simulink model "NBMS_CCCV"  (R2026b)
settings: Solver=FixedStepDiscrete  StopTime=25  FixedStep=0.1
undefined symbols (not defined in the file): CAL_CC_END_DEBOUNCE_TIMER, CAL_CC_END_THRSH, CAL_CHRG_CC_CURRENT_LIMIT, CAL_CHRG_CV_CURRENT_LIMIT, CAL_CHRG_VOLT_LIMIT, CAL_CV_COMPLETE_TIMER, CAL_CV_END_DEBOUNCE_TIMER, CAL_CV_END_THRSH, CAL_CV_WAIT_TIMER, CAL_DD_REVIVAL_CCL, X_CCL_CONT_SAFETY_PACK, Y_CCL_CONT_SAFETY_PACK
settings Model: Creator=hp  LastModifiedBy=rathi
settings OptimizationCC: DefaultParameterBehavior=Inlined  DifferentSizesBufferReuse=on  EfficientTunableParamExpr=on  EnhancedBackFolding=on  OptimizationCustomize=off  OptimizeBlockOrder=speed  PassReuseOutputArgsAs=Individual arguments  RemoveInternalMemoryZeroInit=on  RemoveRootLevelIOMemoryZeroInit=on
settings DebuggingCC: ParameterTunabilityLossMsg=error
settings SFSimCC: MATLABDynamicMemAlloc=off
settings RTWCC: Description=Embedded Coder  GenCodeOnly=on  PackageGeneratedCodeAndArtifacts=on  SystemTargetFile=ert.tlc  TemplateMakefile=ert_default_tmf
settings CodeAppCC: ForceParamTrailComments=on  IgnoreCustomStorageClasses=off  InsertBlockDesc=on  OperatorAnnotations=on  SFDataObjDesc=on  SimulinkDataObjDesc=on
settings ERTTargetCC: DynamicArrayContainerType=coder::array  GenerateSampleERTMain=on
settings ConfigComp: DVDefectChecker=on  DVDetectOutOfBounds=on  DVHarnessSource=Signal Editor  DVModelReferenceHarness=on  DVTestSuiteOptimization=Auto

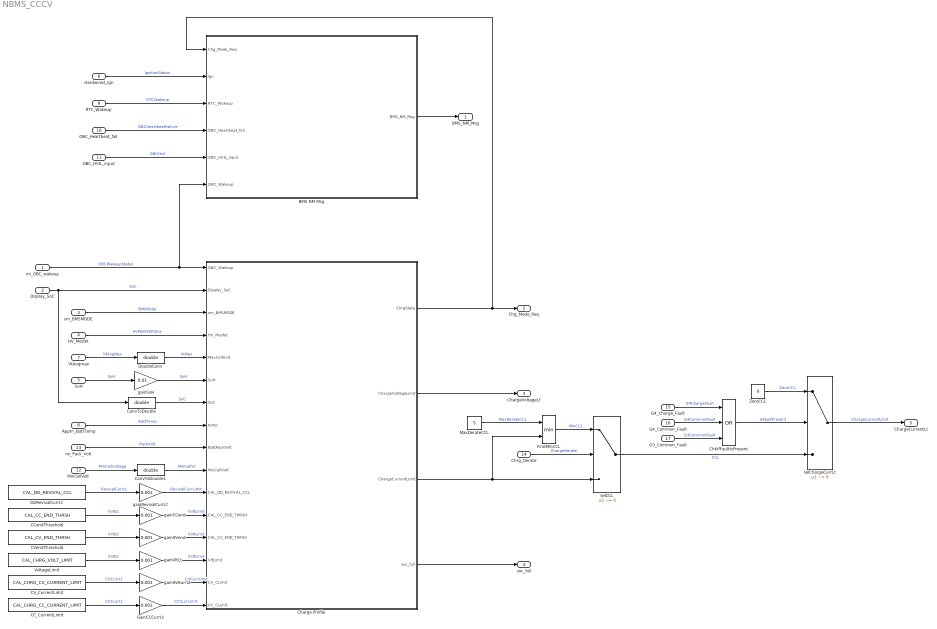
== system NBMS_CCCV ==
  mi_OBC_wakeup : Inport  OutDataTypeStr=Enum: OBC_E
  Display_SoC : Inport  Port=2  OutDataTypeStr=uint8
  sm_BMSMODE : Inport  Port=3  OutDataTypeStr=Enum: BMS_MODE_E
  HV_Mosfet : Inport  Port=4  OutDataTypeStr=Enum: BMS_HVMosfet_STS_E
  SoH : Inport  Port=5  OutDataTypeStr=double
  AppIn_BattTemp : Inport  Port=6  OutDataTypeStr=double
  VtAvgmax : Inport  Port=7  OutDataTypeStr=fixdt(1,16,0.001,0)
  Hardwired_Ign : Inport  Port=8  OutDataTypeStr=boolean
  RTC_Wakeup : Inport  Port=9  OutDataTypeStr=boolean
  OBC_Heartbeat_fail : Inport  Port=10  OutDataTypeStr=boolean
  OBC_HVIL_input : Inport  Port=11  OutDataTypeStr=boolean
  MinCellVolt : Inport  Port=12  OutDataTypeStr=fixdt(1,16,0.001,0)
  mi_Pack_Volt : Inport  Port=13  OutDataTypeStr=double
  Chrg_Derate : Inport  Port=14  OutDataTypeStr=boolean
  G4_Charge_Fault : Inport  Port=15  OutDataTypeStr=boolean
  G4_Common_Fault : Inport  Port=16  OutDataTypeStr=boolean
  G3_Common_Fault : Inport  Port=17  OutDataTypeStr=boolean
  BMS NM Msg : Stateflow chart  TreatAsAtomicUnit=on
      settings: PortSchema="{\"entries\":[{\"content\":{\"sides\":[{\"content\":{\"connectorIds\":[\"In1\",\"In2\",\"In3\",\"In5\",\"In6\",\"In4\"]},\"type\":\"ConnectorPlacement.EquallySpacedRectSide\",\"uuid\":\"e6ae22f8-5427-4fcf-97e7-049847468580\"},{\"content\":{\"connectorIds\":[\"Out1\"],\"side\":\"RIGHT\"},\"type\":\"ConnectorPlacement.EquallySpacedRectSide\",\"uuid\":\"de67337b-b27c-48bc-b99a-9da25b5b262a\"},{\"content\":{\"side\":\"TOP\"},\"type\":\"ConnectorPlacement.EquallySpacedRectSide\",\"uuid\":\"908dc17d-6a46-4063-b5b5-053b8a862aa1\"}]},\"type\":\"ConnectorPlacement.EquallySpacedConnector\",\"uuid\":\"98f653a1-f845-4486-9ef2-8f5f239fd3bd\"}],\"packageUris\":[\"http://schema.mathworks.com/mf0/Connector/R2020b\"],\"version\":\"1.0\"}"
  CC_CurrentLimit : Constant  Value=CAL_CHRG_CC_CURRENT_LIMIT  OutDataTypeStr=double
  CCendThreshold : Constant  Value=CAL_CC_END_THRSH  OutDataTypeStr=double
  CV_CurrentLimit : Constant  Value=CAL_CHRG_CV_CURRENT_LIMIT  OutDataTypeStr=double
  CVendThreshold : Constant  Value=CAL_CV_END_THRSH  OutDataTypeStr=double
  Charge Profile : Stateflow chart  TreatAsAtomicUnit=on
      settings: PortSchema="{\"entries\":[{\"content\":{\"sides\":[{\"content\":{\"connectorIds\":[\"In1\",\"In2\",\"In3\",\"In4\",\"In5\",\"In9\",\"In10\",\"In11\",\"In12\",\"In13\",\"In14\",\"In15\",\"In16\",\"In6\",\"In7\",\"In8\"]},\"type\":\"ConnectorPlacement.EquallySpacedRectSide\",\"uuid\":\"e5a95523-0704-46d3-a42b-abb9c1bf6c2f\"},{\"content\":{\"connectorIds\":[\"Out1\",\"Out2\",\"Out3\",\"Out4\"],\"side\":\"RIGHT\"},\"type\":\"ConnectorPlacement.EquallySpacedRectSide\",\"uuid\":\"018763cc-d3f2-45da-a9d5-aba2061a0002\"},{\"content\":{\"side\":\"TOP\"},\"type\":\"ConnectorPlacement.EquallySpacedRectSide\",\"uuid\":\"2f65ad76-9203-4036-a944-9a805df99265\"}]},\"type\":\"ConnectorPlacement.EquallySpacedConnector\",\"uuid\":\"de439d47-e598-49e1-b63b-f9557df5885d\"}],\"packageUris\":[\"http://schema.mathworks.com/mf0/Connector/R2020b\"],\"version\":\"1.0\"}"
  ChkIfFaultIsPresent : Logic  Operator=OR  Inputs=3  AllPortsSameDT=off  OutDataTypeStr=boolean
  ConvToDouble : DataTypeConversion  OutDataTypeStr=double  SaturateOnIntegerOverflow=off  RndMeth=Floor
  ConvToDouble1 : DataTypeConversion  OutDataTypeStr=double  SaturateOnIntegerOverflow=off  RndMeth=Floor
  DDRevivalCurrLt : Constant  Value=CAL_DD_REVIVAL_CCL  OutDataTypeStr=double
  DoubleConv : DataTypeConversion  OutDataTypeStr=double  SaturateOnIntegerOverflow=off  RndMeth=Floor
  FindMinCCL : MinMax  Inputs=2
  GainCCCurrLt : Gain  Gain=0.001  OutDataTypeStr=double
  MaxDerateCCL : Constant  Value=5  OutDataTypeStr=double
  VoltageLimit : Constant  Value=CAL_CHRG_VOLT_LIMIT  OutDataTypeStr=double
  ZeroCCL : Constant  Value=0  OutDataTypeStr=double
  gainCCend : Gain  Gain=0.001  OutDataTypeStr=double
  gainCVCurrLt : Gain  Gain=0.001  OutDataTypeStr=double
  gainCVend : Gain  Gain=0.001  OutDataTypeStr=double
  gainRevivalCurrLt : Gain  Gain=0.001  OutDataTypeStr=double
  gainSoH : Gain  Gain=0.01  OutDataTypeStr=double
  gainVltLt : Gain  Gain=0.001  OutDataTypeStr=double
  selCCL : Switch  Criteria=u2 ~= 0  SaturateOnIntegerOverflow=off  InputSameDT=off
  selChargeCurrLt : Switch  Criteria=u2 ~= 0  SaturateOnIntegerOverflow=off  InputSameDT=off
  BMS_NM_Msg : Outport
  Chg_Mode_Req : Outport  Port=2  OutDataTypeStr=Enum: Charger_Mode_Req_E
  ChargeVoltageLt : Outport  Port=3  OutDataTypeStr=double
  soc_full : Outport  Port=4  OutDataTypeStr=uint8
  ChargeCurrentLt : Outport  Port=5  OutDataTypeStr=double
  wires:
  mi_OBC_wakeup/1 -> BMS NM Msg/4(OBC_Wakeup), Charge Profile/1(OBC_Wakeup)  "OBCWakeupStatus"
  sm_BMSMODE/1 -> Charge Profile/3(sm_BMSMODE)  "BMSMode"
  HV_Mosfet/1 -> Charge Profile/4(HV_Mosfet)  "HvMosfetStatus"
  VtAvgmax/1 -> DoubleConv/1  "VtAvgMax"
  SoH/1 -> gainSoH/1  "SoH"
  AppIn_BattTemp/1 -> Charge Profile/11(temp)  "BattTemp"
  ConvToDouble/1 -> Charge Profile/10(SoC)  "SoC"
  gainVltLt/1 -> Charge Profile/6(VltLimit)  "VoltLimit"
  VoltageLimit/1 -> gainVltLt/1  "VoltLt"
  gainCVCurrLt/1 -> Charge Profile/7(CV_CLimit)  "CVCurrLimit"
  CV_CurrentLimit/1 -> gainCVCurrLt/1  "CVCurrLt"
  GainCCCurrLt/1 -> Charge Profile/8(CC_CLimit)  "CCCurrLimit"
  CC_CurrentLimit/1 -> GainCCCurrLt/1  "CCCurrLt"
  Charge Profile/1(ChrgState) -> BMS NM Msg/1(Chg_Mode_Req), Chg_Mode_Req/1
  Charge Profile/2(ChargeVoltageLimit) -> ChargeVoltageLt/1
  Charge Profile/3(ChargeCurrentLimit) -> FindMinCCL/2, selCCL/3
  Charge Profile/4(soc_full) -> soc_full/1
  DoubleConv/1 -> Charge Profile/5(MaxCellVolt)  "VtMax"
  Hardwired_Ign/1 -> BMS NM Msg/2(Ign)  "IgnitionStatus"
  RTC_Wakeup/1 -> BMS NM Msg/3(RTC_Wakeup)  "RTCWakeup"
  OBC_Heartbeat_fail/1 -> BMS NM Msg/5(OBC_Heartbeat_fail)  "OBCHeartbeatFailure"
  OBC_HVIL_input/1 -> BMS NM Msg/6(OBC_HVIL_input)  "OBCHvil"
  BMS NM Msg/1(BMS_NM_Msg) -> BMS_NM_Msg/1
  MinCellVolt/1 -> ConvToDouble1/1  "MinCellVoltage"
  mi_Pack_Volt/1 -> Charge Profile/12(BattPackVolt)  "PackVolt"
  ConvToDouble1/1 -> Charge Profile/13(MinCellVolt)  "MinCellVt"
  gainRevivalCurrLt/1 -> Charge Profile/14(CAL_DD_REVIVAL_CCL)  "RevivalCurrLimit"
  DDRevivalCurrLt/1 -> gainRevivalCurrLt/1  "RevivalCurrLt"
  Display_SoC/1 -> ConvToDouble/1, Charge Profile/2(Display_SoC)  "SoC"
  Chrg_Derate/1 -> selCCL/2  "ChargeDerate"
  FindMinCCL/1 -> selCCL/1  "MinCCL"
  MaxDerateCCL/1 -> FindMinCCL/1  "MaxDerateCCL"
  G4_Charge_Fault/1 -> ChkIfFaultIsPresent/1  "G4ChargeFault"
  ZeroCCL/1 -> selChargeCurrLt/1  "ZeroCCL"
  ChkIfFaultIsPresent/1 -> selChargeCurrLt/2  "IsFaultPresent"
  G4_Common_Fault/1 -> ChkIfFaultIsPresent/2  "G4CommonFault"
  selChargeCurrLt/1 -> ChargeCurrentLt/1  "ChargeCurrentLimit"
  G3_Common_Fault/1 -> ChkIfFaultIsPresent/3  "G3CommonFault"
  selCCL/1 -> selChargeCurrLt/3  "CCL"
  CCendThreshold/1 -> gainCCend/1  "VoltLt"
  gainCCend/1 -> Charge Profile/15(CAL_CC_END_THRSH)  "VoltLimit"
  gainCVend/1 -> Charge Profile/16(CAL_CV_END_THRSH)  "VoltLimit"
  CVendThreshold/1 -> gainCVend/1  "VoltLt"
  gainSoH/1 -> Charge Profile/9(SoH)  "SoH"

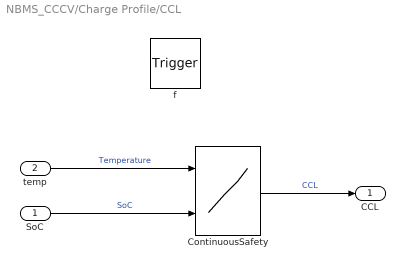
== system NBMS_CCCV/Charge Profile/CCL ==
  SoC : Inport  OutDataTypeStr=double  PortDimensions=1
  temp : Inport  Port=2  OutDataTypeStr=double  PortDimensions=1
  f : TriggerPort  TriggerType=function-call  VariantControl=(inherit)
      settings: CopyFcn=Stateflow.SLINSF.SimulinkMan.removeBlockPreDeleteFcn  PreDeleteFcn=Stateflow.SLINSF.SimulinkMan.unsafePredeleteFcn
  ContinuousSafety : Lookup_n-D  BreakpointsForDimension1=X_CCL_CONT_SAFETY_PACK  BreakpointsForDimension2=Y_CCL_CONT_SAFETY_PACK  Table=[0 0 0 0 0 0 0 0 0 0 0 0 0; 0 0 0 0 0 0 0 0 0 0 0 0 0; 16 16 16 16 3 3 2 2 0 0 0 0 0; 16 16 16 16 7 7 4 4 3 3 2 0 0; 16 16 16 16 16 16 16 16 16 16 16 7 2; 16 16 16 16 16 16 16 16 16 16 16 7 2; 16 16 16 16 16 16 16 16 16 16 16 7 2; 16 16 16 16 16 16 16 16 16 16 16 7 2; 0 0 0 0 0 0 0 0 0 0 0 0 0];  InternalRulePriority=Speed  RndMeth=Simplest
      settings: InputPortMap=u0,u1
  CCL : Outport
  wires:
  SoC/1 -> ContinuousSafety/2  "SoC"
  temp/1 -> ContinuousSafety/1  "Temperature"
  ContinuousSafety/1 -> CCL/1  "CCL"

== stateflow chart NBMS_CCCV/BMS NM Msg ==
  state SLEEP
    en:
    BMS_NM_Msg = BMS_NM_Msg_E.SLEEP;
  state ACTIVE
    en:
    BMS_NM_Msg = BMS_NM_Msg_E.ACTIVE;
  (default) -> SLEEP
  ACTIVE -> SLEEP : [duration(Ign==false && (OBC_HVIL_input==false || ...
      | OBC_Heartbeat_fail ==true || OBC_Wakeup ~= OBC_E.Wake_Up ||...
      | Chg_Mode_Req == Charger_Mode_Req_E.Charge_Complete) &&...
      | RTC_Wakeup == false , sec) >= CAL_NM_MSG_Sleep_timer]
  SLEEP -> ACTIVE : [hasChangedTo(Ign,true) || ...
      | (OBC_HVIL_input == true && RTC_Wakeup == true) || ...
      | (OBC_Heartbeat_fail ==false && hasChangedTo(OBC_Wakeup,OBC_E.Wake_Up))]
  data: Chg_Mode_Req input; Ign input; BMS_NM_Msg output; RTC_Wakeup input; OBC_Wakeup input; OBC_Heartbeat_fail input; OBC_HVIL_input input; CAL_NM_MSG_Sleep_timer parameter

== stateflow chart NBMS_CCCV/Charge Profile ==
  state CHARGE_CCCV
    state Charge_Disable
      en:
      ChrgState = Charger_Mode_Req_E.Disabled;
      ChargeCurrentLimit = 0;
      ChargeVoltageLimit = 0;
      soc_full=0;
    state CV
      en,du:
      ChrgState = Charger_Mode_Req_E.CV;
      ChargeCurrentLimit = CV_CLimit * SoH;
      ChargeVoltageLimit = VltLimit;
    state Charge_Standby
      en:
      ChrgState = Charger_Mode_Req_E.Standby;
      ChargeCurrentLimit = 0;
      ChargeVoltageLimit = 0;
    state CC
      state CC_Start
        en,du:
        ChrgState = Charger_Mode_Req_E.CC_Start;
        ChargeCurrentLimit = CAL_DD_REVIVAL_CCL;
        ChargeVoltageLimit = VltLimit;
        if (BattPackVolt >= 60)
        ChargeCurrentLimit = min(CC_CLimit, CCL(SoC,temp) * SoH);
        ChargeVoltageLimit = VltLimit;
        end
      state CC_End
        en:
        ChrgState = Charger_Mode_Req_E.CC_End;
        ChargeCurrentLimit = 0;
        ChargeVoltageLimit = 0;
      (default) -> CC_Start
      CC_Start -> CC_End : [duration(MaxCellVolt >= CAL_CC_END_THRSH) > CAL_CC_END_DEBOUNCE_TIMER]
    state Charge_Complete
      en:
      ChrgState = Charger_Mode_Req_E.Charge_Complete;
      ChargeCurrentLimit = 0;
      ChargeVoltageLimit = 0;
      soc_full=100;
    (default) -> Charge_Disable
    Charge_Disable -> (junction 68) [order 1] : [Display_SoC == 100]
    (junction 68) -> Charge_Complete
    CV -> Charge_Disable [order 2] : [sm_BMSMODE ~= BMS_MODE_E.BMS_CHARGE]
    CC -> Charge_Disable : [sm_BMSMODE ~= BMS_MODE_E.BMS_CHARGE]
    Charge_Standby -> Charge_Disable [order 3] : [OBC_Wakeup == OBC_E.Sleep]
    Charge_Disable -> (junction 100) [order 2]
    (junction 102) -> (junction 100)
    (junction 100) -> Charge_Standby : [sm_BMSMODE == BMS_MODE_E.BMS_CHARGE && ...
        | OBC_Wakeup == OBC_E.Wake_Up && Display_SoC <= 99 && MinCellVolt >= 2.25]
    Charge_Complete -> (junction 102) : [duration(Display_SoC ~= 100) > 0.2]
    Charge_Standby -> CV [order 2] : [sm_BMSMODE == BMS_MODE_E.BMS_CHARGE && ...
        | HV_Mosfet == BMS_HVMosfet_STS_E.HV_CONNECTED && ...
        | MaxCellVolt >= CAL_CC_END_THRSH]
    Charge_Standby -> CC [order 1] : [sm_BMSMODE == BMS_MODE_E.BMS_CHARGE && ...
        | HV_Mosfet == BMS_HVMosfet_STS_E.HV_CONNECTED && ...
        | MaxCellVolt < CAL_CC_END_THRSH]
    CC_End -> CV : [after(CAL_CV_WAIT_TIMER,sec)]
    CV -> Charge_Complete [order 1] : [duration(MaxCellVolt >= CAL_CV_END_THRSH) > CAL_CV_END_DEBOUNCE_TIMER ||...
        |  after(CAL_CV_COMPLETE_TIMER,sec)]
  state CCL = CCL(SoC,temp) [function]
  data: SoC function_input double size=1; temp function_input double size=1; CCL function_output; ChrgState output; ChargeVoltageLimit output; ChargeCurrentLimit output; OBC_Wakeup input; Display_SoC input; sm_BMSMODE input; HV_Mosfet input; MaxCellVolt input; VltLimit input; CV_CLimit input; CC_CLimit input; SoH input; SoC input; temp input; soc_full output uint8; CAL_CC_END_DEBOUNCE_TIMER parameter; CAL_CV_COMPLETE_TIMER parameter; CAL_CV_END_DEBOUNCE_TIMER parameter; CAL_CV_WAIT_TIMER parameter; BattPackVolt input; MinCellVolt input; CAL_DD_REVIVAL_CCL input; CAL_CC_END_THRSH input; CAL_CV_END_THRSH input
